simulink model "single_phase_multilevel_sm"  (R2026a)
settings: Solver=ode1be  StopTime=simlength  FixedStep=tc
values from neighbouring files (symbols this model uses):
  Vfc1_base = Udc/5    [plotting_modulation.m]    (also in plotting_results.m; plotting_results_hf.m)
  Vfc2_base = 2*Vfc1_base    [plotting_modulation.m]    (also in plotting_results.m; plotting_results_hf.m)
  Vfc3_base = 3*Vfc1_base    [plotting_modulation.m]    (also in plotting_results.m; plotting_results_hf.m)
  Vfc4_base = 4*Vfc1_base    [plotting_modulation.m]    (also in plotting_results.m; plotting_results_hf.m)
undefined symbols (not defined in the file or in its folder): g0_4Hz, g1_4Hz, I_FS, kalman_omega, kalman_theta, ki_i_inv, ki_v_inv, kp_i_inv, kp_v_inv, Lconn, LFu1, m_dead_time, m_duty_open_loop, magnitude, n1, n10, omega_ref, phase_shift_mod11, phase_shift_mod21, phase_shift_mod31, phase_shift_mod41, phase_shift_mod51, precharge_off, q1kalman, q2kalman, Rbalance, Rconn, RFu, Rkalman, RLFu1, tc, time_pwm_enable, tPWM, ts, V_FS, VCFc_5_init, Vgate_base
libraries: fl_lib x103, nesl_utility x61, simulink x1
(part 3 of 3)

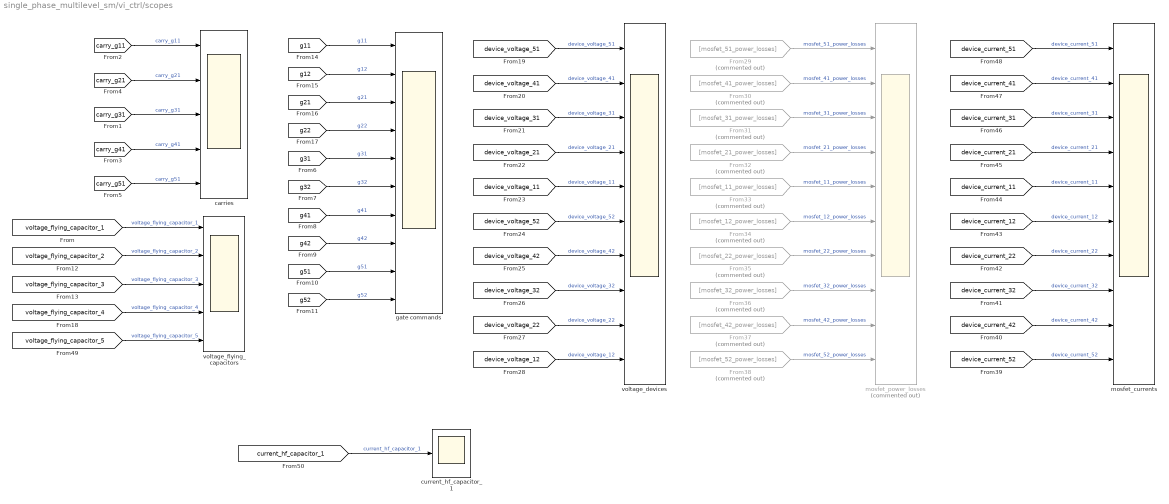
== system single_phase_multilevel_sm/vi_ctrl/scopes ==
  From29 : From  Commented=on  GotoTag=mosfet_51_power_losses
  From30 : From  Commented=on  GotoTag=mosfet_41_power_losses
  From31 : From  Commented=on  GotoTag=mosfet_31_power_losses
  From32 : From  Commented=on  GotoTag=mosfet_21_power_losses
  From33 : From  Commented=on  GotoTag=mosfet_11_power_losses
  From34 : From  Commented=on  GotoTag=mosfet_12_power_losses
  From35 : From  Commented=on  GotoTag=mosfet_22_power_losses
  From36 : From  Commented=on  GotoTag=mosfet_32_power_losses
  From37 : From  Commented=on  GotoTag=mosfet_42_power_losses
  From38 : From  Commented=on  GotoTag=mosfet_52_power_losses
  carries : Scope  NumInputPorts=5
      settings: SampleTime=tc  ActiveDisplayYMinimum=-1.64662  ActiveDisplayYMaximum=1.23308  DataLoggingVariableName=ScopeData2
  current_hf_capacitor_1 : Scope
      settings: SampleTime=tc  ActiveDisplayYMinimum=-3.192455025047797  ActiveDisplayYMaximum=2.3538130408116107
  gate commands : Scope  NumInputPorts=10
      settings: SampleTime=tc  ActiveDisplayYMinimum=-1.875  ActiveDisplayYMaximum=16.875  DataLoggingVariableName=ScopeData3
  mosfet_currents : Scope  NumInputPorts=10
      settings: SampleTime=tc  ActiveDisplayYMinimum=-13.253293794615697  ActiveDisplayYMaximum=13.253429007406689
  mosfet_power_losses : Scope  Commented=on  NumInputPorts=10
      settings: SampleTime=tc  ActiveDisplayYMinimum=-1  ActiveDisplayYMaximum=1  DataLoggingVariableName=ScopeData2
  voltage_devices : Scope  NumInputPorts=10
      settings: SampleTime=tc  ActiveDisplayYMinimum=-91.058092101349729  ActiveDisplayYMaximum=819.44357498501211  DataLoggingVariableName=ScopeData3
  voltage_flying_capacitors : Scope  NumInputPorts=5
      settings: SampleTime=tc  ActiveDisplayYMinimum=239.66616299166378  ActiveDisplayYMaximum=3362.8035828212323
  wires:
  [carry_g51] -> carries/5  "carry_g51"
  [g12] -> gate commands/2  "g12"
  [g11] -> gate commands/1  "g11"
  [g41] -> gate commands/7  "g41"
  [carry_g41] -> carries/4  "carry_g41"
  [g52] -> gate commands/10  "g52"
  [carry_g31] -> carries/3  "carry_g31"
  [g31] -> gate commands/5  "g31"
  [g21] -> gate commands/3  "g21"
  [voltage_flying_capacitor_4] -> voltage_flying_capacitors/4  "voltage_flying_capacitor_4"
  [carry_g11] -> carries/1  "carry_g11"
  [g42] -> gate commands/8  "g42"
  [voltage_flying_capacitor_1] -> voltage_flying_capacitors/1  "voltage_flying_capacitor_1"
  [g22] -> gate commands/4  "g22"
  [g32] -> gate commands/6  "g32"
  [g51] -> gate commands/9  "g51"
  [voltage_flying_capacitor_3] -> voltage_flying_capacitors/3  "voltage_flying_capacitor_3"
  [voltage_flying_capacitor_2] -> voltage_flying_capacitors/2  "voltage_flying_capacitor_2"
  [carry_g21] -> carries/2  "carry_g21"
  [device_current_11] -> mosfet_currents/5  "device_current_11"
  From34/1 -> mosfet_power_losses/6  "mosfet_12_power_losses"
  [device_current_32] -> mosfet_currents/8  "device_current_32"
  From32/1 -> mosfet_power_losses/4  "mosfet_21_power_losses"
  [device_voltage_42] -> voltage_devices/7  "device_voltage_42"
  [device_voltage_21] -> voltage_devices/4  "device_voltage_21"
  [device_current_12] -> mosfet_currents/6  "device_current_12"
  [device_voltage_52] -> voltage_devices/6  "device_voltage_52"
  [device_voltage_41] -> voltage_devices/2  "device_voltage_41"
  [device_voltage_51] -> voltage_devices/1  "device_voltage_51"
  [device_voltage_11] -> voltage_devices/5  "device_voltage_11"
  From31/1 -> mosfet_power_losses/3  "mosfet_31_power_losses"
  [device_voltage_22] -> voltage_devices/9  "device_voltage_22"
  [device_current_51] -> mosfet_currents/1  "device_current_51"
  [device_current_41] -> mosfet_currents/2  "device_current_41"
  [device_voltage_12] -> voltage_devices/10  "device_voltage_12"
  [device_voltage_32] -> voltage_devices/8  "device_voltage_32"
  [device_voltage_31] -> voltage_devices/3  "device_voltage_31"
  From36/1 -> mosfet_power_losses/8  "mosfet_32_power_losses"
  From33/1 -> mosfet_power_losses/5  "mosfet_11_power_losses"
  From29/1 -> mosfet_power_losses/1  "mosfet_51_power_losses"
  From30/1 -> mosfet_power_losses/2  "mosfet_41_power_losses"
  From37/1 -> mosfet_power_losses/9  "mosfet_42_power_losses"
  From38/1 -> mosfet_power_losses/10  "mosfet_52_power_losses"
  From35/1 -> mosfet_power_losses/7  "mosfet_22_power_losses"
  [device_current_42] -> mosfet_currents/9  "device_current_42"
  [device_current_31] -> mosfet_currents/3  "device_current_31"
  [device_current_22] -> mosfet_currents/7  "device_current_22"
  [device_current_21] -> mosfet_currents/4  "device_current_21"
  [device_current_52] -> mosfet_currents/10  "device_current_52"
  [voltage_flying_capacitor_5] -> voltage_flying_capacitors/5  "voltage_flying_capacitor_5"
  [current_hf_capacitor_1] -> current_hf_capacitor_1/1  "current_hf_capacitor_1"

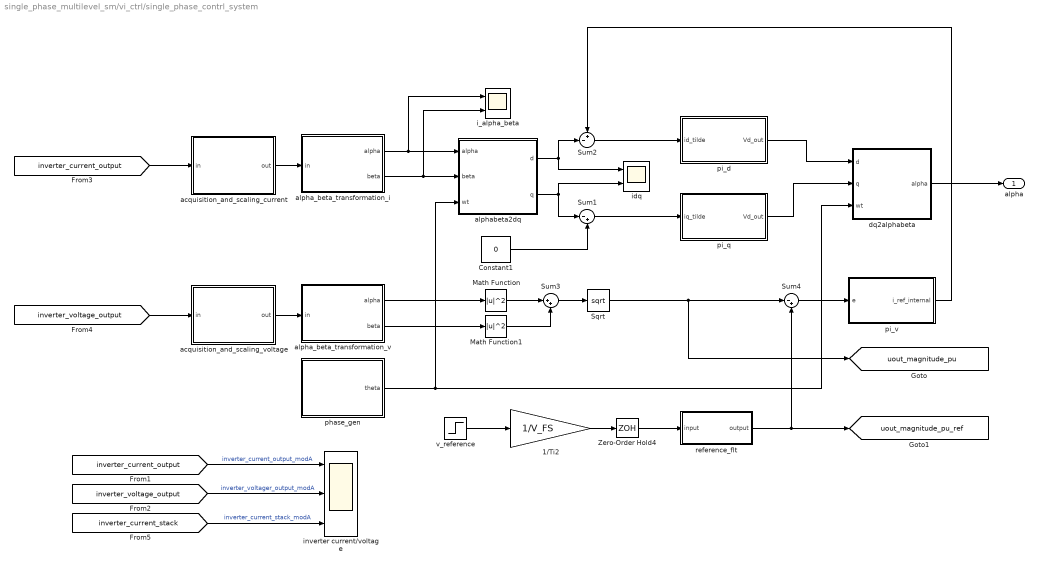
== system single_phase_multilevel_sm/vi_ctrl/single_phase_contrl_system ==
  1/Ti2 : Gain  Gain=1/V_FS  SaturateOnIntegerOverflow=on  OutDataTypeStr=Inherit: Same as input  ParamDataTypeStr=Inherit: Same as input
  Constant1 : Constant  Value=0
  Math Function : Math  Operator=magnitude^2
  Math Function1 : Math  Operator=magnitude^2
  Sqrt : Sqrt
  Sum1 : Sum  Inputs=|-+
  Sum2 : Sum  Inputs=+-|
  Sum3 : Sum  Inputs=|++
  Sum4 : Sum  Inputs=|-+
  Zero-Order Hold4 : ZeroOrderHold  SampleTime=ts
  acquisition_and_scaling_current : Subsystem
  acquisition_and_scaling_voltage : Subsystem
  alpha_beta_transformation_i : Subsystem
  alpha_beta_transformation_v : Subsystem
  alphabeta2dq : Subsystem
  dq2alphabeta : Subsystem
  i_alpha_beta : Scope  NumInputPorts=2
      settings: ActiveDisplayYMinimum=-8.21139788811583E-18  ActiveDisplayYMaximum=9.9342010258853445E-18
  idq : Scope  NumInputPorts=2
      settings: ActiveDisplayYMinimum=-0.09367  ActiveDisplayYMaximum=0.50142
  inverter current/voltage : Scope  NumInputPorts=3
      settings: SampleTime=tc  ActiveDisplayYMinimum=-5.781446495004932  ActiveDisplayYMaximum=5.8368797471135245  DataLoggingVariableName=ScopeData2
  phase_gen : Subsystem
  pi_d : Subsystem
  pi_q : Subsystem
  pi_v : Subsystem
  reference_flt : Subsystem
  v_reference : Step  Time=precharge_off  FinalValue=230*sqrt(2)  SampleTime=0
  alpha : Outport
  tag scope: uout_magnitude_pu=global, uout_magnitude_pu_ref=global
  wires:
  [inverter_current_output] -> inverter current/voltage/1  "inverter_current_output_modA"
  [inverter_current_output] -> acquisition_and_scaling_current/1(in)
  pi_d/1(Vd_out) -> dq2alphabeta/1(d)
  pi_v/1(i_ref_internal) -> Sum2/1
  Zero-Order Hold4/1 -> reference_flt/1(input)
  alpha_beta_transformation_v/2(beta) -> Math Function1/1
  [inverter_voltage_output] -> inverter current/voltage/2  "inverter_voltager_output_modA"
  alphabeta2dq/2("q ") -> idq/2, Sum1/1
  dq2alphabeta/1(alpha) -> alpha/1
  [inverter_voltage_output] -> acquisition_and_scaling_voltage/1(in)
  Constant1/1 -> Sum1/2
  alphabeta2dq/1("d ") -> idq/1, Sum2/2
  v_reference/1 -> 1/Ti2/1
  Sum4/1 -> pi_v/1(e)
  Math Function1/1 -> Sum3/2
  phase_gen/1(theta) -> alphabeta2dq/3(wt), dq2alphabeta/3(wt)
  1/Ti2/1 -> Zero-Order Hold4/1
  acquisition_and_scaling_current/1(out) -> alpha_beta_transformation_i/1(in)
  Sum3/1 -> Sqrt/1
  Sum1/1 -> pi_q/1(iq_tilde)
  Math Function/1 -> Sum3/1
  Sqrt/1 -> [uout_magnitude_pu], Sum4/1
  pi_q/1(Vd_out) -> dq2alphabeta/2(q)
  Sum2/1 -> pi_d/1(id_tilde)
  alpha_beta_transformation_i/1(alpha) -> i_alpha_beta/1, alphabeta2dq/1(alpha)
  alpha_beta_transformation_i/2(beta) -> i_alpha_beta/2, alphabeta2dq/2(beta)
  acquisition_and_scaling_voltage/1(out) -> alpha_beta_transformation_v/1(in)
  alpha_beta_transformation_v/1(alpha) -> Math Function/1
  [inverter_current_stack] -> inverter current/voltage/3  "inverter_current_stack_modA"
  reference_flt/1(output) -> [uout_magnitude_pu_ref], Sum4/2

== system single_phase_multilevel_sm/output_filter/instantaneus_power/mavg_1 ==
  in : Inport
  Gain : Gain  Gain=n1-1
  Gain1 : Gain  Gain=1/n1
  Sum : Sum  Inputs=|++
  Unit Delay : UnitDelay  SampleTime=ts
  out : Outport  VectorParamsAs1DForOutWhenUnconnected=off
  wires:
  Sum/1 -> Gain1/1
  Unit Delay/1 -> Gain/1
  in/1 -> Sum/1
  Gain1/1 -> out/1, Unit Delay/1
  Gain/1 -> Sum/2

== system single_phase_multilevel_sm/output_filter/instantaneus_power/rms2 ==
  vout : Inport
  Gain : Gain  Gain=n10-1
  Gain1 : Gain  Gain=1/n10
  Math Function : Math  Operator=magnitude^2  SignedPower=on
  Sqrt : Sqrt
  Sum : Sum  Inputs=|++
  Unit Delay : UnitDelay  SampleTime=ts
  Out1 : Outport  VectorParamsAs1DForOutWhenUnconnected=off
  wires:
  vout/1 -> Math Function/1
  Sum/1 -> Gain1/1
  Gain1/1 -> Sqrt/1, Unit Delay/1
  Unit Delay/1 -> Gain/1
  Math Function/1 -> Sum/1
  Sqrt/1 -> Out1/1
  Gain/1 -> Sum/2

== system single_phase_multilevel_sm/output_filter/instantaneus_power/rms3 ==
  iout : Inport
  Gain : Gain  Gain=n10-1
  Gain1 : Gain  Gain=1/n10
  Math Function : Math  Operator=magnitude^2  SignedPower=on
  Sqrt : Sqrt
  Sum : Sum  Inputs=|++
  Unit Delay : UnitDelay  SampleTime=ts
  Out1 : Outport  VectorParamsAs1DForOutWhenUnconnected=off
  wires:
  Gain/1 -> Sum/2
  Sqrt/1 -> Out1/1
  Math Function/1 -> Sum/1
  Unit Delay/1 -> Gain/1
  Gain1/1 -> Unit Delay/1, Sqrt/1
  Sum/1 -> Gain1/1
  iout/1 -> Math Function/1

== system single_phase_multilevel_sm/vi_ctrl/modulator1/triangle_1 ==
  Constant : Constant  Value=pi/2
  Product : Product  Inputs=*/
  Sine Wave : Sin  Frequency=2*pi/tPWM  Phase=phase_shift_mod11  SampleTime=0
  Trigonometric Function : Trigonometry  Operator=asin
  carry_mod11 : Outport
  wires:
  Constant/1 -> Product/2
  Sine Wave/1 -> Trigonometric Function/1
  Trigonometric Function/1 -> Product/1
  Product/1 -> carry_mod11/1

== system single_phase_multilevel_sm/vi_ctrl/modulator2/triangle_1 ==
  Constant : Constant  Value=pi/2
  Product : Product  Inputs=*/
  Sine Wave : Sin  Frequency=2*pi/tPWM  Phase=phase_shift_mod21  SampleTime=0
  Trigonometric Function : Trigonometry  Operator=asin
  carry_mod21 : Outport
  wires:
  Trigonometric Function/1 -> Product/1
  Sine Wave/1 -> Trigonometric Function/1
  Constant/1 -> Product/2
  Product/1 -> carry_mod21/1

== system single_phase_multilevel_sm/vi_ctrl/modulator3/triangle_1 ==
  Constant : Constant  Value=pi/2
  Product : Product  Inputs=*/
  Sine Wave : Sin  Frequency=2*pi/tPWM  Phase=phase_shift_mod31  SampleTime=0
  Trigonometric Function : Trigonometry  Operator=asin
  carry_mod21 : Outport
  wires:
  Product/1 -> carry_mod21/1
  Constant/1 -> Product/2
  Sine Wave/1 -> Trigonometric Function/1
  Trigonometric Function/1 -> Product/1

== system single_phase_multilevel_sm/vi_ctrl/modulator4/triangle_1 ==
  Constant : Constant  Value=pi/2
  Product : Product  Inputs=*/
  Sine Wave : Sin  Frequency=2*pi/tPWM  Phase=phase_shift_mod41  SampleTime=0
  Trigonometric Function : Trigonometry  Operator=asin
  carry_mod21 : Outport
  wires:
  Product/1 -> carry_mod21/1
  Constant/1 -> Product/2
  Sine Wave/1 -> Trigonometric Function/1
  Trigonometric Function/1 -> Product/1

== system single_phase_multilevel_sm/vi_ctrl/modulator5/triangle_1 ==
  Constant : Constant  Value=pi/2
  Product : Product  Inputs=*/
  Sine Wave : Sin  Frequency=2*pi/tPWM  Phase=phase_shift_mod51  SampleTime=0
  Trigonometric Function : Trigonometry  Operator=asin
  carry_mod21 : Outport
  wires:
  Trigonometric Function/1 -> Product/1
  Sine Wave/1 -> Trigonometric Function/1
  Constant/1 -> Product/2
  Product/1 -> carry_mod21/1

== system single_phase_multilevel_sm/vi_ctrl/single_phase_contrl_system/acquisition_and_scaling_current ==
  in : Inport
  1/Ti5 : Gain  Gain=1/I_FS  SaturateOnIntegerOverflow=on  OutDataTypeStr=Inherit: Same as input  ParamDataTypeStr=Inherit: Same as input
  Unit Delay4 : UnitDelay  SampleTime=ts
  Zero-Order Hold1 : ZeroOrderHold  SampleTime=ts
  out : Outport
  wires:
  in/1 -> Zero-Order Hold1/1
  1/Ti5/1 -> Unit Delay4/1
  Zero-Order Hold1/1 -> 1/Ti5/1
  Unit Delay4/1 -> out/1

== system single_phase_multilevel_sm/vi_ctrl/single_phase_contrl_system/acquisition_and_scaling_voltage ==
  in : Inport
  1/Ti1 : Gain  Gain=1/V_FS  SaturateOnIntegerOverflow=on  OutDataTypeStr=Inherit: Same as input  ParamDataTypeStr=Inherit: Same as input
  Unit Delay4 : UnitDelay  SampleTime=ts
  Zero-Order Hold2 : ZeroOrderHold  SampleTime=ts
  out : Outport
  wires:
  1/Ti1/1 -> Unit Delay4/1
  Zero-Order Hold2/1 -> 1/Ti1/1
  Unit Delay4/1 -> out/1
  in/1 -> Zero-Order Hold2/1

== system single_phase_multilevel_sm/vi_ctrl/single_phase_contrl_system/alpha_beta_transformation_i ==
  in : Inport
  Constant1 : Constant  Value=omega_ref
  Constant3 : Constant  Value=q1kalman
  Constant4 : Constant  Value=q2kalman
  Constant5 : Constant  Value=Rkalman
  Constant6 : Constant  Value=ts
  Gain : Gain  Gain=-1
  kalman_observer : MATLAB Function  TreatAsAtomicUnit=on  SystemSampleTime=ts
  alpha : Outport
  beta : Outport  Port=2
  wires:
  Constant4/1 -> kalman_observer/5(q2)
  Constant3/1 -> kalman_observer/4(q1)
  Constant5/1 -> kalman_observer/6(r)
  Constant6/1 -> kalman_observer/3(Ts)
  in/1 -> kalman_observer/1(y)
  Constant1/1 -> kalman_observer/2(w)
  kalman_observer/2(h2_hat) -> Gain/1
  kalman_observer/1(h1_hat) -> alpha/1
  Gain/1 -> beta/1

== system single_phase_multilevel_sm/vi_ctrl/single_phase_contrl_system/alpha_beta_transformation_v ==
  in : Inport
  Constant1 : Constant  Value=omega_ref
  Constant3 : Constant  Value=q1kalman
  Constant4 : Constant  Value=q2kalman
  Constant5 : Constant  Value=Rkalman
  Constant6 : Constant  Value=ts
  Gain : Gain  Gain=-1
  kalman_observer : MATLAB Function  TreatAsAtomicUnit=on  SystemSampleTime=ts
  alpha : Outport
  beta : Outport  Port=2
  wires:
  Gain/1 -> beta/1
  kalman_observer/1(h1_hat) -> alpha/1
  kalman_observer/2(h2_hat) -> Gain/1
  Constant1/1 -> kalman_observer/2(w)
  in/1 -> kalman_observer/1(y)
  Constant6/1 -> kalman_observer/3(Ts)
  Constant5/1 -> kalman_observer/6(r)
  Constant3/1 -> kalman_observer/4(q1)
  Constant4/1 -> kalman_observer/5(q2)

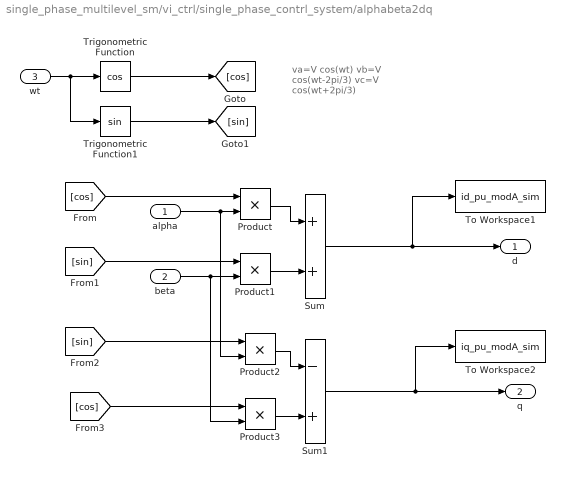
== system single_phase_multilevel_sm/vi_ctrl/single_phase_contrl_system/alphabeta2dq ==
  note: va=V cos(wt)
      | vb=V cos(wt-2pi/3)
      | vc=V cos(wt+2pi/3)
  alpha : Inport
  beta : Inport  Port=2
  wt : Inport  Port=3
  Product{,1..3} (4 alike) : Product  RndMeth=Zero
  Sum : Sum
  Sum1 : Sum  Inputs=-+
  To Workspace1 : ToWorkspace  VariableName=id_pu_modA_sim  SampleTime=ts
      settings: MaxDataPoints=Ns
  To Workspace2 : ToWorkspace  VariableName=iq_pu_modA_sim  SampleTime=ts
      settings: MaxDataPoints=Ns
  Trigonometric Function : Trigonometry  Operator=cos
  Trigonometric Function1 : Trigonometry
  "d " : Outport  VectorParamsAs1DForOutWhenUnconnected=off
  "q " : Outport  Port=2  VectorParamsAs1DForOutWhenUnconnected=off
  wires:
  wt/1 -> Trigonometric Function1/1, Trigonometric Function/1
  Trigonometric Function/1 -> [cos]
  Trigonometric Function1/1 -> [sin]
  [cos] -> Product/1
  alpha/1 -> Product/2, Product2/2
  Product/1 -> Sum/1
  Product1/1 -> Sum/2
  [sin] -> Product1/1
  beta/1 -> Product1/2, Product3/2
  Sum/1 -> To Workspace1/1, "d "/1
  [sin] -> Product2/1
  Product2/1 -> Sum1/1
  Product3/1 -> Sum1/2
  [cos] -> Product3/1
  Sum1/1 -> To Workspace2/1, "q "/1

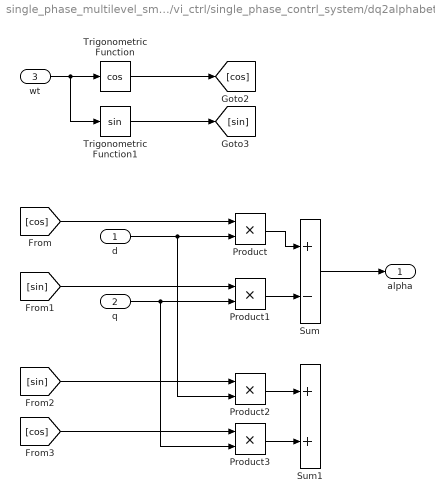
== system single_phase_multilevel_sm/vi_ctrl/single_phase_contrl_system/dq2alphabeta ==
  d : Inport
  q : Inport  Port=2
  wt : Inport  Port=3
  Product{,1..3} (4 alike) : Product  RndMeth=Zero
  Sum : Sum  Inputs=+-
  Sum1 : Sum
  Trigonometric Function : Trigonometry  Operator=cos
  Trigonometric Function1 : Trigonometry
  alpha : Outport  VectorParamsAs1DForOutWhenUnconnected=off
  wires:
  [cos] -> Product3/1
  Product3/1 -> Sum1/2
  Product2/1 -> Sum1/1
  [sin] -> Product2/1
  Sum/1 -> alpha/1
  q/1 -> Product3/2, Product1/2
  [sin] -> Product1/1
  Product1/1 -> Sum/2
  Product/1 -> Sum/1
  d/1 -> Product2/2, Product/2
  [cos] -> Product/1
  Trigonometric Function1/1 -> [sin]
  Trigonometric Function/1 -> [cos]
  wt/1 -> Trigonometric Function/1, Trigonometric Function1/1

== system single_phase_multilevel_sm/vi_ctrl/single_phase_contrl_system/phase_gen ==
  load_estimator : Subsystem
  signal_generator : Subsystem
  theta : Outport
  wires:
  signal_generator/1(theta) -> theta/1

== system single_phase_multilevel_sm/vi_ctrl/single_phase_contrl_system/pi_d ==
  id_tilde : Inport
  1/Ti : Gain  Gain=kp_i_inv  SaturateOnIntegerOverflow=on  OutDataTypeStr=Inherit: Same as input  ParamDataTypeStr=Inherit: Same as input
  Sum1 : Sum  Inputs=+++  SaturateOnIntegerOverflow=on
  Sum3 : Sum  Inputs=-+  SaturateOnIntegerOverflow=on
  To Workspace3 : ToWorkspace  VariableName=id_ctrl_out_modA_sim  SampleTime=ts
      settings: MaxDataPoints=Ns
  Unit Delay4 : UnitDelay  SampleTime=ts
  kp2 : Gain  Gain=ki_i_inv*ts  SaturateOnIntegerOverflow=on  OutDataTypeStr=Inherit: Same as input  ParamDataTypeStr=Inherit: Same as input
  ud_out_lim : Saturate  UpperLimit=1  LowerLimit=-1
  Vd_out : Outport  VectorParamsAs1DForOutWhenUnconnected=off
  wires:
  id_tilde/1 -> kp2/1, 1/Ti/1
  Sum1/1 -> ud_out_lim/1
  kp2/1 -> Sum1/2
  1/Ti/1 -> Sum1/1, Sum3/1
  Unit Delay4/1 -> Sum1/3
  Sum3/1 -> Unit Delay4/1
  ud_out_lim/1 -> To Workspace3/1, Vd_out/1, Sum3/2

== system single_phase_multilevel_sm/vi_ctrl/single_phase_contrl_system/pi_q ==
  iq_tilde : Inport
  1/Ti : Gain  Gain=kp_i_inv  SaturateOnIntegerOverflow=on  OutDataTypeStr=Inherit: Same as input  ParamDataTypeStr=Inherit: Same as input
  Sum1 : Sum  Inputs=+++  SaturateOnIntegerOverflow=on
  Sum3 : Sum  Inputs=-+  SaturateOnIntegerOverflow=on
  To Workspace3 : ToWorkspace  VariableName=iq_ctrl_out_modA_sim  SampleTime=ts
      settings: MaxDataPoints=Ns
  Unit Delay4 : UnitDelay  SampleTime=ts
  kp2 : Gain  Gain=ki_i_inv*ts  SaturateOnIntegerOverflow=on  OutDataTypeStr=Inherit: Same as input  ParamDataTypeStr=Inherit: Same as input
  ud_out_lim : Saturate  UpperLimit=1  LowerLimit=-1
  Vd_out : Outport  VectorParamsAs1DForOutWhenUnconnected=off
  wires:
  ud_out_lim/1 -> Vd_out/1, To Workspace3/1, Sum3/2
  Sum3/1 -> Unit Delay4/1
  Unit Delay4/1 -> Sum1/3
  1/Ti/1 -> Sum3/1, Sum1/1
  kp2/1 -> Sum1/2
  Sum1/1 -> ud_out_lim/1
  iq_tilde/1 -> 1/Ti/1, kp2/1

== system single_phase_multilevel_sm/vi_ctrl/single_phase_contrl_system/pi_v ==
  e : Inport
  1/Ti : Gain  Gain=kp_v_inv  SaturateOnIntegerOverflow=on  OutDataTypeStr=Inherit: Same as input  ParamDataTypeStr=Inherit: Same as input
  Sum1 : Sum  Inputs=+++  SaturateOnIntegerOverflow=on
  Sum3 : Sum  Inputs=-+  SaturateOnIntegerOverflow=on
  Unit Delay4 : UnitDelay  SampleTime=ts
  i_out_lim : Saturate  UpperLimit=0.869565217391304  LowerLimit=0
  kp2 : Gain  Gain=ki_v_inv*ts  SaturateOnIntegerOverflow=on  OutDataTypeStr=Inherit: Same as input  ParamDataTypeStr=Inherit: Same as input
  i_ref_internal : Outport  VectorParamsAs1DForOutWhenUnconnected=off
  tag scope: inverter_current_reference=global
  wires:
  i_out_lim/1 -> [inverter_current_reference], i_ref_internal/1, Sum3/2
  Sum3/1 -> Unit Delay4/1
  Unit Delay4/1 -> Sum1/3
  1/Ti/1 -> Sum3/1, Sum1/1
  kp2/1 -> Sum1/2
  Sum1/1 -> i_out_lim/1
  e/1 -> kp2/1, 1/Ti/1

== system single_phase_multilevel_sm/vi_ctrl/single_phase_contrl_system/reference_flt ==
  input : Inport
  Gain3 : Gain  Gain=g1_4Hz
  Gain6 : Gain  Gain=g0_4Hz
  Sum : Sum  Inputs=|++
  Unit Delay1 : UnitDelay  SampleTime=ts
  output : Outport  VectorParamsAs1DForOutWhenUnconnected=off
  wires:
  Gain6/1 -> Sum/1
  input/1 -> Gain6/1
  Unit Delay1/1 -> Gain3/1
  Gain3/1 -> Sum/2
  Sum/1 -> Unit Delay1/1, output/1

== system single_phase_multilevel_sm/vi_ctrl/single_phase_contrl_system/phase_gen/load_estimator ==
  theta : Inport
  Gain : Gain  Gain=kalman_omega
  Gain1 : Gain  Gain=kalman_theta
  Gain5 : Gain  Gain=ts
  Sum : Sum  Inputs=-+|
  Sum1 : Sum  Inputs=|++
  Sum2 : Sum  Inputs=|++
  Sum8 : Sum  Inputs=++|
  Unit Delay1 : UnitDelay  SampleTime=ts
  Unit Delay2 : UnitDelay  SampleTime=ts
  bounder1 : MATLAB Function  TreatAsAtomicUnit=on  SystemSampleTime=ts
  bounder2 : MATLAB Function  TreatAsAtomicUnit=on  SystemSampleTime=ts
  theta_hat : Outport  VectorParamsAs1DForOutWhenUnconnected=off
  wires:
  theta/1 -> Sum/2  "theta"
  Sum8/1 -> bounder2/1(u)
  Sum1/1 -> Unit Delay2/1
  Unit Delay2/1 -> Sum1/2, Gain5/1
  Sum2/1 -> Sum8/2
  bounder2/1(y) -> Unit Delay1/1
  bounder1/1(y) -> Gain/1, Gain1/1
  Sum/1 -> bounder1/1(u)
  Unit Delay1/1 -> Sum2/2, theta_hat/1, Sum/1  "theta_hat"
  Gain5/1 -> Sum8/1
  Gain1/1 -> Sum2/1
  Gain/1 -> Sum1/1

== system single_phase_multilevel_sm/vi_ctrl/single_phase_contrl_system/phase_gen/signal_generator ==
  Unit Delay2 : UnitDelay  SampleTime=ts
  signal_generator : Subsystem
  theta : Outport
  wires:
  Unit Delay2/1 -> theta/1
  signal_generator/1(theta) -> Unit Delay2/1

== system single_phase_multilevel_sm/vi_ctrl/single_phase_contrl_system/phase_gen/signal_generator/signal_generator ==
  Constant4 : Constant  Value=omega_ref
  Constant7 : Constant
  Product2 : Product  RndMeth=Zero
  Sum4 : Sum  SaturateOnIntegerOverflow=on
  Unit Delay1 : UnitDelay  SampleTime=ts
  bounder : MATLAB Function  TreatAsAtomicUnit=on  SystemSampleTime=ts
  kp2 : Gain  Gain=ts  SaturateOnIntegerOverflow=on  OutDataTypeStr=Inherit: Same as input  ParamDataTypeStr=Inherit: Same as input
  theta : Outport
  wires:
  Product2/1 -> kp2/1
  bounder/1(y) -> Unit Delay1/1, theta/1
  kp2/1 -> Sum4/1
  Constant7/1 -> Product2/1
  Constant4/1 -> Product2/2
  Unit Delay1/1 -> Sum4/2
  Sum4/1 -> bounder/1(u)

== matlab function single_phase_multilevel_sm/vi_ctrl/single_phase_contrl_system/alpha_beta_transformation_v/kalman_observer ==
  data: y input; h1_hat output; w input; Ts input; q1 input; q2 input; r input; h2_hat output
function [h1_hat, h2_hat]   = KFO(y,w,Ts,q1,q2,r)

    persistent   x1_po x2_po p11_po p12_po p21_po p22_po

    if isempty(x1_po)
        x1_po = 0;
        x2_po = 0;
        p11_po = 0;
        p12_po = 0;
        p21_po = 0;
        p22_po = 0;        
    end
    
    a11 = cos(w*Ts);
    a12 = sin(w*Ts);
    a21 = -sin(w*Ts);
    a22 = cos(w*Ts);
    
    x1_pr = a11*x1_po + a12*x2_po;
    x2_pr = a21*x1_po + a22*x2_po;
    
    p11_pr = q1 + a11*(a11*p11_po+a12*p21_po) + a12*(a11*p12_po+a12*p22_po);
    p12_pr = a21*(a11*p11_po+a12*p21_po) + a22*(a11*p12_po+a12*p22_po);
    p21_pr = a11*(a21*p11_po+a22*p21_po) + a12*(a21*p12_po+a22*p22_po);
    p22_pr = q2 + a21*(a21*p11_po+a22*p21_po) + a22*(a21*p12_po+a22*p22_po);
    
    l1 = p11_pr/(p11_pr + r);
    l2 = p21_pr/(p11_pr + r);
    
    x1_po = x1_pr + l1*(y-x1_pr);
    x2_po = x2_pr + l2*(y-x1_pr);
    
    p11_po = (1-l1)*p11_pr;
    p12_po = (1-l1)*p12_pr;
    p21_po = p21_pr-l2*p11_pr;
    p22_po = p22_pr-l2*p12_pr;
    
    h1_hat = x1_pr;
    h2_hat = x2_pr;
end

== matlab function single_phase_multilevel_sm/vi_ctrl/single_phase_contrl_system/phase_gen/signal_generator/signal_generator/bounder ==
  data: u input; y output
function y = bounder(u)
    
    y = -pi + mod(u+3*pi,2*pi);
   
end

== matlab function single_phase_multilevel_sm/vi_ctrl/single_phase_contrl_system/phase_gen/load_estimator/bounder1 ==
  data: u input; y output
function y = bounder(u)
    
    u = -pi + mod(u+3*pi,2*pi);
    
    y = u;
end

== matlab function single_phase_multilevel_sm/vi_ctrl/single_phase_contrl_system/phase_gen/load_estimator/bounder2 ==
  data: u input; y output
function y = bounder(u)
    
    u = -pi + mod(u+3*pi,2*pi);
    
    y = u;
end

== matlab function single_phase_multilevel_sm/vi_ctrl/single_phase_contrl_system/alpha_beta_transformation_i/kalman_observer ==
  data: y input; h1_hat output; w input; Ts input; q1 input; q2 input; r input; h2_hat output
function [h1_hat, h2_hat]   = KFO(y,w,Ts,q1,q2,r)

    persistent   x1_po x2_po p11_po p12_po p21_po p22_po

    if isempty(x1_po)
        x1_po = 0;
        x2_po = 0;
        p11_po = 0;
        p12_po = 0;
        p21_po = 0;
        p22_po = 0;        
    end
    
    a11 = cos(w*Ts);
    a12 = sin(w*Ts);
    a21 = -sin(w*Ts);
    a22 = cos(w*Ts);
    
    x1_pr = a11*x1_po + a12*x2_po;
    x2_pr = a21*x1_po + a22*x2_po;
    
    p11_pr = q1 + a11*(a11*p11_po+a12*p21_po) + a12*(a11*p12_po+a12*p22_po);
    p12_pr = a21*(a11*p11_po+a12*p21_po) + a22*(a11*p12_po+a12*p22_po);
    p21_pr = a11*(a21*p11_po+a22*p21_po) + a12*(a21*p12_po+a22*p22_po);
    p22_pr = q2 + a21*(a21*p11_po+a22*p21_po) + a22*(a21*p12_po+a22*p22_po);
    
    l1 = p11_pr/(p11_pr + r);
    l2 = p21_pr/(p11_pr + r);
    
    x1_po = x1_pr + l1*(y-x1_pr);
    x2_po = x2_pr + l2*(y-x1_pr);
    
    p11_po = (1-l1)*p11_pr;
    p12_po = (1-l1)*p12_pr;
    p21_po = p21_pr-l2*p11_pr;
    p22_po = p22_pr-l2*p12_pr;
    
    h1_hat = x1_pr;
    h2_hat = x2_pr;
end
